simulink model "Single_Phase_Vienna_Inverter"  (R2023b)
settings: Solver=VariableStepAuto  StartTime=0.0  StopTime=1  FixedStep=2e-6  RelTol=1e-3
libraries: spsIGBTDiodeLib x8, spsSeriesRLCBranchLib x6, spsVoltageMeasurementLib x4, simulink x2, spsCurrentMeasurementLib x1, spsDCVoltageSourceLib x1, spsMeanLib x1, powerlib_extras x1, spsTHDLib x1, spspowerguiLib x1
settings Model: SimulationMode=accelerator  Creator=abc6820292  LastModifiedBy=c
settings DebuggingCC: UnconnectedInputMsg=warning  UnconnectedOutputMsg=warning  UnconnectedLineMsg=warning
settings ModelReferenceCC: EnableRefExpFcnMdlSchedulingChecks=on
settings RTWCC: DLArmComputeVersion=19.05

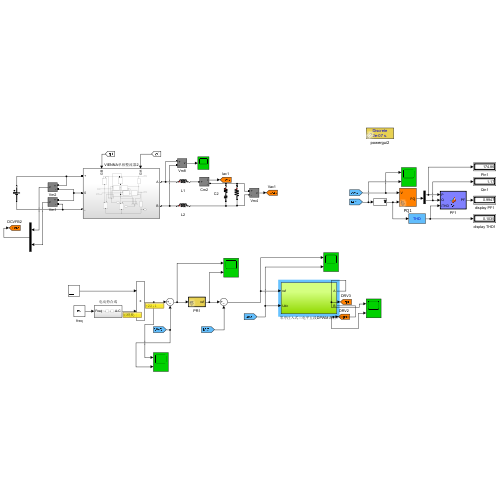
[thumbnail: Simulink's stored preview of the top-level diagram]
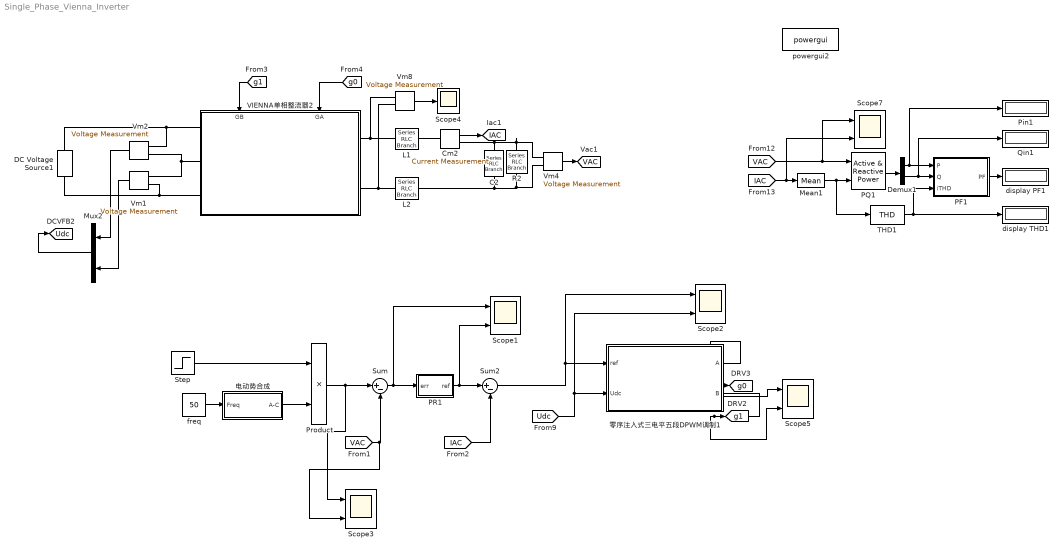
== system Single_Phase_Vienna_Inverter ==
  C2 : spsSeriesRLCBranchLib/Series RLC Branch  LConnTagsString=__new0  RConnTagsString=__new0  BranchType=RC  Resistance=0.01  Inductance=0  SetiL0=off  InitialCurrent=0  Capacitance=2e-6  Setx0=on  InitialVoltage=30  Measurements=None
  Cm2 : spsCurrentMeasurementLib/Current Measurement  PhasorSimulation=off  OutputType=Complex  PSBequivalent=0
  DC Voltage Source1 : spsDCVoltageSourceLib/DC Voltage Source  Amplitude=60  Measurements=None
  Demux1 : Demux  Outputs=2
  L1 : spsSeriesRLCBranchLib/Series RLC Branch  LConnTagsString=__new0  RConnTagsString=__new0  BranchType=L  Resistance=30  Inductance=200e-6  SetiL0=off  InitialCurrent=0  Capacitance=1e-3  Setx0=off  InitialVoltage=0  Measurements=None
  L2 : spsSeriesRLCBranchLib/Series RLC Branch  LConnTagsString=__new0  RConnTagsString=__new0  BranchType=L  Resistance=30  Inductance=200e-6  SetiL0=off  InitialCurrent=0  Capacitance=1e-3  Setx0=off  InitialVoltage=0  Measurements=None
  Mean1 : spsMeanLib/Mean  Freq=16000  Vinit=0  Ts=0
  Mux2 : Mux  Inputs=2
  PF1 : MATLAB Function  TreatAsAtomicUnit=on
  PQ1 : powerlib_extras/Measurements/Active & Reactive Power  f1=50
  PR1 : Subsystem  TreatAsAtomicUnit=on  mask{Kp=1, Kr=100, Wc=5, Upper=1000, Lower=-1000}
  Pin1 : Display
      settings: Format=bank
  Product : Product
  Qin1 : Display
      settings: Format=bank
  R2 : spsSeriesRLCBranchLib/Series RLC Branch  LConnTagsString=__new0  RConnTagsString=__new0  BranchType=R  Resistance=5  Inductance=7e-4  SetiL0=off  InitialCurrent=0  Capacitance=1e-3  Setx0=off  InitialVoltage=0  Measurements=None
  Scope{1..3,5,7} (5 alike) : Scope  NumInputPorts=2
  Scope4 : Scope
  Step : Step  Time=0.2  Before=20*1.414  After=30*1.414  SampleTime=0
  Sum : Sum  Inputs=|+-
  Sum2 : Sum  Inputs=|+-
  THD1 : spsTHDLib/THD  Freq=50  Ts=0
  VIENNA单相整流器2 : Subsystem
      settings: PortSchema="{\"entries\":[{\"content\":{\"sides\":[{\"content\":{\"connectorIds\":[\"LConn1\",\"LConn2\",\"LConn3\"]},\"type\":\"ConnectorPlacement.EquallySpacedRectSide\",\"uuid\":\"47187a24-6853-42ac-9ad9-0df0e1360fae\"},{\"content\":{\"connectorIds\":[\"RConn1\",\"RConn2\"],\"side\":\"RIGHT\"},\"type\":\"ConnectorPlacement.EquallySpacedRectSide\",\"uuid\":\"b3504369-b235-4116-9b9b-167bd6b76527\"},{\"content\":{\"connectorIds\":[\"In1\",\"In2\"],\"side\":\"TOP\"},\"type\":\"ConnectorPlacement.EquallySpacedRectSide\",\"uuid\":\"5cb205b4-da18-4f20-b3d4-22846a9c2236\"},{\"content\":{\"connectorIds\":[],\"side\":\"BOTTOM\"},\"type\":\"ConnectorPlacement.EquallySpacedRectSide\",\"uuid\":\"4e548a82-6bdf-470e-8572-00c7c8855d01\"}]},\"type\":\"ConnectorPlacement.EquallySpacedConnector\",\"uuid\":\"b00ba750-ea4b-4b64-a122-5cbc9e899126\"}],\"packageUris\":[\"http://schema.mathworks.com/mf0/Connector/R2020b\"],\"version\":\"1.0\"}"
  Vm{1..2,4,8} (4 alike) : spsVoltageMeasurementLib/Voltage Measurement  PhasorSimulation=off  OutputType=Complex  PSBequivalent=0
  display PF1 : Display
  display THD1 : Display
  freq : Constant  Value=50
  powergui2 : spspowerguiLib/powergui  SimulationMode=Discrete  SampleTime=2e-7  frequency=60  Iterations=50  frequencyindice=0  Pbase=100e6  ErrMax=1e-4  UnitsV=kV  UnitsW=MW  buscounter=0  FunctionMessages=off  echomessages=off  EnableUseOfTLC=off  CurrentSourceSwitches=off  DisableSnubberDevices=off  DisableRonSwitches=off  DisableVfSwitches=off  DisplayEquations=off  AutomaticDiscreteSolvers=off  SolverType=Tustin/Backward Euler (TBE)  Interpol=off  ExternalGateDelay=off  methode=off  Ts=0  x0status=blocks  SPID=off  SwTol=0  HookPort=off  NonlinearTolerance=1e-4  nMaxIteration=100  ContinueOnMaxIteration=off  RestoreLinks=warning  ResistiveCurrentMeasurement=off  Frange=[0:2:500]  Ylog=off  Xlog=on  ShowGrid=off  save=off  variable=ZData  structure=QQQQQ  ZoomFFT=off  StartTime=0.5  cycles=15  DisplayStyle=1  fundamental=50  FreqAxis=off  MaxFrequency=1000  frequencyindicesteady=1  RmsSteady=1  display=off
  电动势合成 : Subsystem
      settings: PortSchema="{\"entries\":[{\"content\":{\"sides\":[{\"content\":{\"connectorIds\":[]},\"type\":\"ConnectorPlacement.EquallySpacedRectSide\",\"uuid\":\"ac756fcf-f6d7-466d-bb3d-287dec8ae983\"},{\"content\":{\"connectorIds\":[],\"side\":\"RIGHT\"},\"type\":\"ConnectorPlacement.EquallySpacedRectSide\",\"uuid\":\"3e1a0e91-a0b8-40c4-8839-5ebd84050a30\"},{\"content\":{\"connectorIds\":[\"In1\"],\"side\":\"TOP\"},\"type\":\"ConnectorPlacement.EquallySpacedRectSide\",\"uuid\":\"4c3986ff-483b-4975-8d50-1a8a46f35065\"},{\"content\":{\"connectorIds\":[\"Out1\"],\"side\":\"BOTTOM\"},\"type\":\"ConnectorPlacement.EquallySpacedRectSide\",\"uuid\":\"d0166e46-df65-4061-a961-140d500477a7\"}]},\"type\":\"ConnectorPlacement.EquallySpacedConnector\",\"uuid\":\"9d4b00aa-dfb1-427d-8698-7ec64c5ca012\"}],\"packageUris\":[\"http://schema.mathworks.com/mf0/Connector/R2020b\"],\"version\":\"1.0\"}"
  零序注入式三电平五段DPWM调制1 : Subsystem
  tag scope: IAC=global, Udc=global, VAC=global, g0=global, g1=global
  wires:
  freq/1 -> 电动势合成/1(Freq)
  Step/1 -> Product/1
  电动势合成/1(A-C) -> Product/2
  Product/1 -> Scope3/1, Sum/1
  [VAC] -> Scope3/2, Sum/2
  Sum/1 -> Scope1/1, PR1/1(err)
  PR1/1(ref) -> Scope1/2, Sum2/1
  [IAC] -> Sum2/2
  Demux1/1 -> PF1/1(P), Pin1/1
  PF1/1(PF) -> display PF1/1
  [VAC] -> PQ1/1, Scope7/1
  Demux1/2 -> PF1/2(Q), Qin1/1
  [IAC] -> Mean1/1, Scope7/2
  THD1/1 -> PF1/3(iTHD), display THD1/1
  Mean1/1 -> PQ1/2, THD1/1
  PQ1/1 -> Demux1/1
  [Udc] -> Scope2/2, 零序注入式三电平五段DPWM调制1/2(Udc)
  Sum2/1 -> Scope2/1, 零序注入式三电平五段DPWM调制1/1(ref)
  [g0] -> VIENNA单相整流器2/2(GA)
  [g1] -> VIENNA单相整流器2/1(GB)
  Vm8/1 -> Scope4/1
  Vm4/1 -> [VAC]
  Cm2/1 -> [IAC]
  Mux2/1 -> [Udc]
  Vm1/1 -> Mux2/2
  Vm2/1 -> Mux2/1
  零序注入式三电平五段DPWM调制1/1(A) -> Scope5/1, [g0]
  零序注入式三电平五段DPWM调制1/2(B) -> Scope5/2, [g1]
  connections:
  Vm2/LConn1 -- DC Voltage Source1/RConn1 -- VIENNA单相整流器2/LConn1
  Vm1/LConn2 -- DC Voltage Source1/LConn1 -- VIENNA单相整流器2/LConn3
  Vm1/LConn1 -- Vm2/LConn2 -- VIENNA单相整流器2/LConn2
  Vm8/LConn2 -- VIENNA单相整流器2/RConn2 -- L2/LConn1
  L1/LConn1 -- Vm8/LConn1 -- VIENNA单相整流器2/RConn1
  Vm4/LConn1 -- R2/LConn1 -- C2/LConn1 -- Cm2/RConn1
  Vm4/LConn2 -- R2/RConn1 -- C2/RConn1 -- L2/RConn1
  Cm2/LConn1 -- L1/RConn1

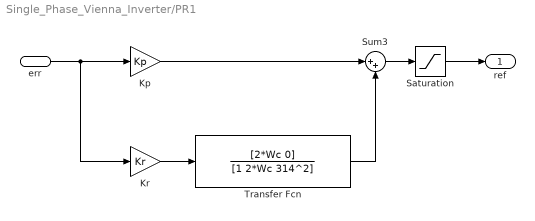
== system Single_Phase_Vienna_Inverter/PR1 ==
  err : Inport
  Kp : Gain  Gain=Kp
  Kr : Gain  Gain=Kr
  Saturation : Saturate  UpperLimit=Upper  LowerLimit=Lower
  Sum3 : Sum  Inputs=|++
  Transfer Fcn : TransferFcn  Numerator=[2*Wc 0]  Denominator=[1 2*Wc 314^2]
  ref : Outport
  wires:
  Saturation/1 -> ref/1
  Transfer Fcn/1 -> Sum3/2
  Kr/1 -> Transfer Fcn/1
  err/1 -> Kp/1, Kr/1
  Sum3/1 -> Saturation/1
  Kp/1 -> Sum3/1

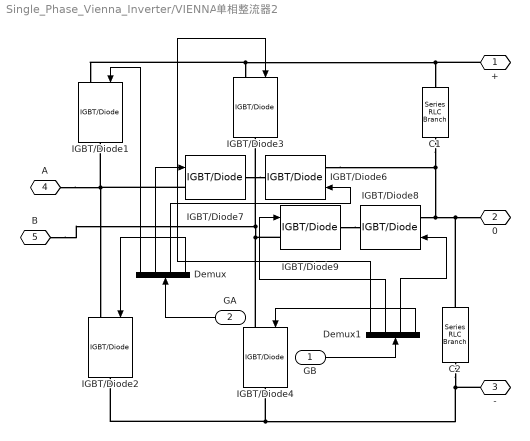
== system Single_Phase_Vienna_Inverter/VIENNA单相整流器2 ==
  GB : Inport
  GA : Inport  Port=2
  C1 : spsSeriesRLCBranchLib/Series RLC Branch  LConnTagsString=__new0  RConnTagsString=__new0  BranchType=RC  Resistance=0.01  Inductance=0  SetiL0=off  InitialCurrent=0  Capacitance=2e-3  Setx0=on  InitialVoltage=30  Measurements=None
  C2 : spsSeriesRLCBranchLib/Series RLC Branch  LConnTagsString=__new0  RConnTagsString=__new0  BranchType=RC  Resistance=0.1  Inductance=0  SetiL0=off  InitialCurrent=0  Capacitance=2e-3  Setx0=on  InitialVoltage=30  Measurements=None
  Demux : Demux
  Demux1 : Demux
  IGBT/Diode{1..4,6..9} (8 alike) : spsIGBTDiodeLib/IGBT//Diode  Ron=1e-3  Rs=1e5  Cs=inf  Measurements=off
  + : PMIOPort  Side=Left
  0 : PMIOPort  Port=2  Side=Left
  - : PMIOPort  Port=3  Side=Left
  A : PMIOPort  Port=4  Side=Right
  B : PMIOPort  Port=5  Side=Right
  wires:
  GA/1 -> Demux/1
  GB/1 -> Demux1/1
  Demux/3 -> IGBT/Diode6/1
  Demux/2 -> IGBT/Diode7/1
  Demux1/3 -> IGBT/Diode8/1
  Demux1/2 -> IGBT/Diode9/1
  Demux/1 -> IGBT/Diode1/1
  Demux/4 -> IGBT/Diode2/1
  Demux1/1 -> IGBT/Diode3/1
  Demux1/4 -> IGBT/Diode4/1
  connections:
  IGBT/Diode3/RConn1 -- B/RConn1 -- IGBT/Diode9/LConn1 -- IGBT/Diode4/LConn1
  +/RConn1 -- IGBT/Diode1/LConn1 -- IGBT/Diode3/LConn1 -- C1/LConn1
  -/RConn1 -- IGBT/Diode2/RConn1 -- IGBT/Diode4/RConn1 -- C2/RConn1
  A/RConn1 -- IGBT/Diode7/LConn1 -- IGBT/Diode1/RConn1 -- IGBT/Diode2/LConn1
  IGBT/Diode7/RConn1 -- IGBT/Diode6/RConn1
  IGBT/Diode8/LConn1 -- C1/RConn1 -- IGBT/Diode6/LConn1 -- C2/LConn1 -- 0/RConn1
  IGBT/Diode9/RConn1 -- IGBT/Diode8/RConn1

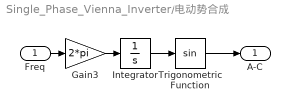
== system Single_Phase_Vienna_Inverter/电动势合成 ==
  Freq : Inport
  Gain3 : Gain  Gain=2*pi
  Integrator : Integrator  WrapState=on  WrappedStateUpperValue=2*pi  WrappedStateLowerValue=0
  Trigonometric Function : Trigonometry
  A-C : Outport
  wires:
  Gain3/1 -> Integrator/1
  Trigonometric Function/1 -> A-C/1
  Integrator/1 -> Trigonometric Function/1
  Freq/1 -> Gain3/1

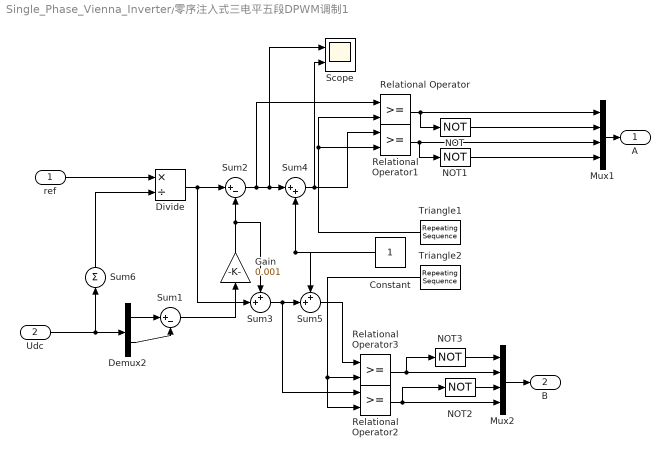
== system Single_Phase_Vienna_Inverter/零序注入式三电平五段DPWM调制1 ==
  ref : Inport
  Udc : Inport  Port=2
  Constant : Constant
  Demux2 : Demux  Outputs=2
  Divide : Product  Inputs=*/
  Gain : Gain  Gain=0.001
  Mux1 : Mux
  Mux2 : Mux
  NOT{,1..3} (4 alike) : Logic  Operator=NOT  IconShape=distinctive  AllPortsSameDT=off  OutDataTypeStr=boolean
  Relational Operator{,1..3} (4 alike) : RelationalOperator  OutDataTypeStr=boolean  InputSameDT=off
  Scope : Scope  NumInputPorts=2
  Sum1 : Sum  Inputs=|+-
  Sum2 : Sum  Inputs=|+-
  Sum3 : Sum  Inputs=++|
  Sum4 : Sum  Inputs=|++
  Sum5 : Sum  Inputs=++|
  Sum6 : Sum  Inputs=+
  Triangle1 : simulink/Sources/Repeating Sequence  rep_seq_t=[0 1/60000/2 1/60000]  rep_seq_y=[0 1 0]
  Triangle2 : simulink/Sources/Repeating Sequence  rep_seq_t=[0 1/60000/2 1/60000]  rep_seq_y=[1 0 1]
  A : Outport
  B : Outport  Port=2
  wires:
  NOT3/1 -> Mux2/1
  NOT2/1 -> Mux2/3
  NOT1/1 -> Mux1/4
  NOT/1 -> Mux1/2
  Triangle2/1 -> Relational Operator3/2, Relational Operator2/2
  Sum6/1 -> Divide/2
  Constant/1 -> Sum5/1, Sum4/2
  Sum5/1 -> Relational Operator3/1
  Relational Operator2/1 -> NOT2/1, Mux2/4
  Relational Operator3/1 -> Mux2/2, NOT3/1
  Triangle1/1 -> Relational Operator1/2, Relational Operator/2
  Sum3/1 -> Sum5/2, Relational Operator2/1
  Sum4/1 -> Scope/2, Relational Operator1/1
  Divide/1 -> Sum2/1, Sum3/2
  Gain/1 -> Sum2/2, Sum3/1
  Mux1/1 -> A/1
  Relational Operator1/1 -> Mux1/3, NOT1/1
  Relational Operator/1 -> NOT/1, Mux1/1
  Mux2/1 -> B/1
  Demux2/2 -> Sum1/2
  Demux2/1 -> Sum1/1
  ref/1 -> Divide/1
  Sum2/1 -> Scope/1, Sum4/1, Relational Operator/1
  Sum1/1 -> Gain/1
  Udc/1 -> Demux2/1, Sum6/1

== matlab function Single_Phase_Vienna_Inverter/PF1 ==
  data: P input; PF output; Q input; iTHD input
function PF = fcn(P,Q,iTHD)
% This block supports an embeddable subset of the MATLAB language.
% See the help menu for details. 
PF=(P/sqrt(P*P+Q*Q))/(sqrt(1+iTHD*iTHD));
